simulink model "Maxom_fcs_noncascaded"  (R2025b)
settings: Solver=ode45  StartTime=0.0  StopTime=0.30  FixedStep=1e-6  MaxStep=1e-5  RelTol=1e-4  EnableMultiTasking=on
values from neighbouring files (symbols this model uses):
  Bfric = 0    [PMSMpara.m]
  ffai = 0.008667    [PMSMpara.m]
  Imax = 20    [PMSMpara.m]
  J = 0.044e-4    (= 4.4e-06)    [PMSMpara.m]
  kis = 0    [PMSMpara.m]
  kps = fsc*6.28*J/Kt    (= 0.364364007978)    [PMSMpara.m]
  Kt = np*1.5*ffai    (= 0.0910035)    [PMSMpara.m]
  Ld = Ls    (= 0.00045)    [PMSMpara.m]
  Lq = Ls    (= 0.00045)    [PMSMpara.m]
  np = 7    [PMSMpara.m]
  Rs = 0.5    [PMSMpara.m]
  Tcur = 1/32000    (= 3.125e-05)    [PMSMpara.m]
  Tpwm = 1/32000    (= 3.125e-05)    [PMSMpara.m]
  Tspd = 1/32000    (= 3.125e-05)    [PMSMpara.m]
  wn = 311040    [PMSMpara.m]
  zeta = 1    [PMSMpara.m]
undefined symbols (not defined in the file or in its folder): dspblkCoreblockFVToolHelper, gcbh
libraries: simulink x4, slpidlib x2, spsUniversalBridgeLib x1, spsCurrentMeasurementLib x1, EasyGo_Machine_lib x1, spsPermanentMagnetSynchronousMachineLib x1, spsSVPWMGenerator2LevelLib x1, spsDCVoltageSourceLib x1, sps_lib x1
(part 1 of 4)
Description:
  | %20230207 r13c
  | 版本同 servo_32k_TSMI_r12b_0413ff02mv8_4t9c2cnst
  | 负载转矩前馈滤波截止频率提到1500hz
  | 
  | r13d  模型版本等同 servo_32k_TSMI_r12b_0413ff02mv8_4t11b2
  | 修改速度给定滤波处理逻辑
  | 小改转矩前馈控制系数
settings Model: ModifiedComment=danie -- Wed Jan 05 16:58:37 2022 -- Version 1.4214  ParamWorkspaceSource=ReferencedWorkspace  TunableVars=Comp_curr_lmt,CurrRampTime_s,DT_Comp_curr_lmt,DT_Comp_curr_uplmt,DT_Comp_freq_lmt,DT_Comp_freq_lmt1,DT_Comp_freq_off_lmt,DT_Comp_reg_uplmt,DT_Comp_table_length,DeadTime_comp_mode,DecOVPEn,K_angle_comp,K_obs,Ki_udcctrl_ID,Kp_udcctrl_ID,Kudcctrl,OpenLoopCtrlEn,OvIdLmtMax,OvIdLmtMin,OverVoltLmHi,SPD_RES_EN,Servo_start_mode,SynFailCfmTime_ms,SynFailDetectEnable,Udc,We_Adapt_Max_set,damping_enable,dc_pos_time,dt_comp_curr_table,dt_comp_reg_table,flystr_sc_time,fs_flystart_Hz_set,fw_us_max,idc_pos_ref,idc_pos_time,iq_opnlp_curr_ref,is_opn_max,k_TorqFwd_c1,k_TorqFwd_c2,k_aw,k_emf_cnst_krpm,k_load_torq_comp,k_res_damp1,k_res_damp2,k_we_damp,k_wr_adj,ki_cur_ctrl,ki_flux_wkn,ki_is_load_comp,ki_is_magn_comp,ki_psir_adapt,ki_rs_adapt,ki_spd_ctrl,ki_spd_ctrl_low,ki_we_adapt,ki_wr_est_pll,kp_cur_ctrl,kp_flux_wkn,kp_is_load_comp,kp_is_magn_comp,kp_psir_adapt,kp_rs_adapt,kp_spd_ctrl,kp_spd_ctrl_low,kp_we_adapt,kp_wr_est_pll,ld_calc,lq_calc,maxfreqref_Hz,motor_start_mode,mtr_rated_cur_set,mtr_rated_freq_set,normal_acc_time_s,openloopTest,opnlp_acc_time,pn_calc,psir_calc,rs_calc,sc_test_Imax,spd_ctrl_out_max,spd_ctrl_out_min,startfrqholdtime_s,sw_wr_hi,sw_wr_lo,sw_wr_mag_hi,sw_wr_mag_lo,swtich_freq_spd_ctrl_hi,swtich_freq_spd_ctrl_low,ts_calc_cur_set,ts_calc_obs_set,ts_flystart_set,udc_r,ukf_spd_calc_en,w_startfrq,ws_merge_mode,ws_no_merge  TunableVarsStorageClass=Auto,Auto,Auto,Auto,Auto,Auto,Auto,Auto,Auto,Auto,Auto,Auto,Auto,Auto,Auto,Auto,Auto,Auto,Auto,Auto,Auto,Auto,Auto,Auto,Auto,Auto,Auto,Auto,Auto,Auto,Auto,Auto,Auto,Auto,Auto,Auto,Auto,Auto,Auto,Auto,Auto,Auto,Auto,Auto,Auto,Auto,Auto,Auto,Auto,Auto,Auto,Auto,Auto,Auto,Auto,Auto,Auto,Auto,Auto,Auto,Auto,Auto,Auto,Auto,Auto,Auto,Auto,Auto,Auto,Auto,Auto,Auto,Auto,Auto,Auto,Auto,Auto,Auto,Auto,Auto,Auto,Auto,Auto,Auto,Auto,Auto,Auto,Auto,Auto,Auto,Auto,Auto,Auto,Auto,Auto,Auto  TunableVarsTypeQualifier=,,,,,,,,,,,,,,,,,,,,,,,,,,,,,,,,,,,,,,,,,,,,,,,,,,,,,,,,,,,,,,,,,,,,,,,,,,,,,,,,,,,,,,,,,,,,,,,  VariantFading=off  Creator=MATLAB05  LastModifiedBy=dayanakhegay
settings Model: ModifiedHistory=|
  | danie -- Wed Jan 05 16:58:37 2022 -- Version 1.4214
  | 
  | 
  | danie -- Wed Jan 05 16:58:37 2022 -- Version 1.4214
  | 
  | 
  | danie -- Wed Jan 05 16:44:40 2022 -- Version 1.4213
  | 
  | 
  | danie -- Wed Jan 05 16:23:23 2022 -- Version 1.4212
  | 
  | 
  | danie -- Wed Jan 05 15:12:40 2022 -- Version 1.4211
  | 
  | 
  | danie -- Wed Jan 05 11:32:37 2022 -- Version 1.4208
  | 
  | 
  | danie -- Wed Jan 05 11:32:37 2022 -- Version 1.4208
  | 
  | 
  | danie -- Wed Jan 05 11:32:37 2022 -- Version 1.4208
  | 
  | 
  | danie -- Wed Jan 05 11:32:37 2022 -- Version 1.4208
  | 
  | 
  | danie -- Wed Jan 05 11:32:37 2022 -- Version 1.4208
  | 
  | 
  | danie -- Wed Jan 05 11:32:37 2022 -- Version 1.4208
  | 
  | 
  | danie -- Wed Jan 05 11:32:37 2022 -- Version 1.4208
  | 
  | 
  | danie -- Wed Jan 05 11:32:37 2022 -- Version 1.4208
  | 
  | 
  | danie -- Tue Jan 04 20:01:11 2022 -- Version 1.4189
  | 
  | 
  | danie -- Tue Jan 04 20:01:11 2022 -- Version 1.4189
  | 
  | 
  | danie -- Tue Jan 04 20:01:11 2022 -- Version 1.4189
  | 
  | 
  | danie -- Tue Jan 04 20:01:11 2022 -- Version 1.4189
  | 
  | 
  | danie -- Tue Jan 04 20:01:11 2022 -- Version 1.4189
  | 
  | 
  | danie -- Tue Jan 04 20:01:11 2022 -- Version 1.4189
  | 
  | 
  | danie -- Tue Jan 04 20:01:11 2022 -- Version 1.4189
  | 
  | 
  | danie -- Tue Jan 04 20:01:11 2022 -- Version 1.4189
  | 
  | 
  | danie -- Tue Jan 04 20:01:11 2022 -- Version 1.4189
  | 
  | 
  | danie -- Tue Jan 04 20:01:11 2022 -- Version 1.4189
  | 
  | 
  | danie -- Tue Jan 04 20:01:11 2022 -- Version 1.4189
  | 
  | 
  | danie -- Tue Jan 04 20:01:11 2022 -- Version 1.4189
  | 
  | 
  | danie -- Tue Jan 04 20:01:11 2022 -- Version 1.4189
  | 
  | 
  | danie -- Tue Jan 04 20:01:11 2022 -- Version 1.4189
  | 
  | 
  | danie -- Tue Jan 04 20:01:11 2022 -- Version 1.4189
  | 
  | 
  | danie -- Tue Jan 04 20:01:11 2022 -- Version 1.4189
  | 
  | 
  | danie -- Tue Jan 04 20:01:11 2022 -- Version 1.4189
  | 
  | 
  | danie -- Tue Jan 04 20:01:11 2022 -- Version 1.4189
  | 
  | 
  | danie -- Tue Jan 04 20:01:11 2022 -- Version 1.4189
  | 
  | 
  | danie -- Tue Jan 04 20:01:11 2022 -- Version 1.4189
  | 
  | 
  | danie -- Tue Jan 04 20:01:11 2022 -- Version 1.4189
  | 
  | 
  | danie -- Tue Jan 04 20:01:11 2022 -- Version 1.4189
  | 
  | 
  | danie -- Tue Jan 04 20:01:11 2022 -- Version 1.4189
  | 
  | 
  | danie -- Tue Jan 04 20:01:11 2022 -- Version 1.4189
  | 
  | 
  | danie -- Tue Jan 04 20:01:11 2022 -- Version 1.4189
  | 
  | 
  | danie -- Tue Jan 04 20:01:11 2022 -- Version 1.4189
  | 
  | 
  | danie -- Tue Jan 04 20:01:11 2022 -- Version 1.4189
  | 
  | 
  | danie -- Tue Jan 04 20:01:11 2022 -- Version 1.4189
  | 
  | 
  | danie -- Tue Jan 04 20:01:11 2022 -- Version 1.4189
  | 
  | 
  | danie -- Tue Jan 04 20:01:11 2022 -- Version 1.4189
  | 
  | 
  | danie -- Tue Jan 04 20:01:11 2022 -- Version 1.4189
  | 
  | 
  | danie -- Tue Jan 04 18:06:07 2022 -- Version 1.4188
  | 
  | 
  | danie -- Tue Jan 04 17:34:36 2022 -- Version 1.4187
  | 
  | 
  | danie -- Tue Jan 04 17:26:52 2022 -- Version 1.4186
  | 
  | 
  | danie -- Tue Jan 04 17:22:15 2022 -- Version 1.4185
  | add merge mode 2( time merge mode)
  | 
  | danie -- Tue Jan 04 16:56:47 2022 -- Version 1.4179
  | 
  | 
  | danie -- Tue Jan 04 16:56:47 2022 -- Version 1.4179
  | 
  | 
  | danie -- Tue Jan 04 16:56:47 2022 -- Version 1.4179
  | 
  | 
  | danie -- Tue Jan 04 16:56:47 2022 -- Version 1.4179
  | 
  | 
  | danie -- Tue Jan 04 16:56:47 2022 -- Version 1.4179
  | 
  | 
  | danie -- Tue Jan 04 16:56:47 2022 -- Version 1.4179
  | 
  | 
  | danie -- Tue Jan 04 16:56:47 2022 -- Version 1.4179
  | 
  | 
  | danie -- Tue Jan 04 16:56:47 2022 -- Version 1.4179
  | 
  | 
  | danie -- Tue Jan 04 16:24:52 2022 -- Version 1.4174
  | 
  | 
  | danie -- Tue Jan 04 16:24:52 2022 -- Version 1.4174
  | 
  | 
  | danie -- Tue Jan 04 16:24:52 2022 -- Version 1.4174
  | 
  | 
  | danie -- Tue Jan 04 16:24:52 2022 -- Version 1.4174
  | 
  | 
  | danie -- Tue Jan 04 16:24:52 2022 -- Version 1.4174
  | 
  | 
  | danie -- Tue Jan 04 16:24:52 2022 -- Version 1.4174
  | 
  | 
  | danie -- Tue Jan 04 16:13:51 2022 -- Version 1.4173
  | 
  | try to modify merge（low/high spd）spd fdb logic
  | 
  | danie -- Tue Jan 04 15:54:14 2022 -- Version 1.4172
  | 
  | 
  | danie -- Thu Dec 30 11:22:47 2021 -- Version 1.4171
  | 
  | 
  | danie -- Thu Dec 30 11:13:03 2021 -- Version 1.4170
  | 
  | 
  | danie -- Thu Dec 30 10:44:02 2021 -- Version 1.4167
  | 
  | 
  | danie -- Thu Dec 30 10:44:02 2021 -- Version 1.4167
  | 
  | 
  | danie -- Thu Dec 30 10:44:02 2021 -- Version 1.4167
  | 
  | 
  | danie -- Thu Dec 30 10:37:28 2021 -- Version 1.4166
  | 
  | 
  | danie -- Wed Dec 29 18:47:50 2021 -- Version 1.4165
  | 
  | 
  | danie -- Wed Dec 29 18:47:08 2021 -- Version 1.4164
  | 
  | 优化转矩前馈，和电流指令前馈
  | 修改速度PID模块，
  | 速度环输出加入超前滞后补偿环节
  | 
  | danie -- Tue Dec 28 11:57:05 2021 -- Version 1.4144
  | 
  | 1. fix alig function logic， function code write-back logic debug
  | 2. dec run logic after 2-levle current control（10hz），
  | 3. save eeprom ok
settings SolverCC: AlgebraicLoopSolver=TrustRegion
settings DataIOCC: LimitDataPoints=on  SaveFormat=StructureWithTime  SignalLoggingSaveFormat=ModelDataLogs  DSMLogging=off  ReturnWorkspaceOutputs=off
settings OptimizationCC: DefaultParameterBehavior=Inlined  UseFloatMulNetSlope=on  DefaultUnderspecifiedDataType=single  UseSpecifiedMinMax=on  InlineInvariantSignals=on  ExpressionDepthLimit=2147483647.0  StateBitsets=on  DataBitsets=on  ZeroExternalMemoryAtStartup=off  InitFltsAndDblsToZero=on  EfficientFloat2IntCast=on  EfficientMapNaN2IntZero=off  LifeSpan=1  SimCompilerOptimization=on  EfficientTunableParamExpr=on
settings DebuggingCC: SignalInfNanChecking=warning  SignalRangeChecking=warning  SaveWithParameterizedLinksMsg=none  UnderspecifiedInitializationDetection=Classic  MergeDetectMultiDrivingBlocksExec=none  SignalResolutionControl=TryResolveAllWithWarning  MaxConsecutiveZCsMsg=none  SolverPrmCheckMsg=warning  CheckMatrixSingularityMsg=warning  ParameterPrecisionLossMsg=none  ParameterTunabilityLossMsg=none  UnconnectedInputMsg=warning  UnconnectedOutputMsg=warning  UnconnectedLineMsg=warning  AllowSymbolicDim=off  StateNameClashWarn=warning  SFUnexpectedBacktrackingDiag=warning  SFNoUnconditionalDefaultTransitionDiag=warning  SFExecutionAtInitializationDiag=none  ArithmeticOperatorsInVariantConditions=warning
settings HardwareCC: ProdBitPerPointer=32.0  ProdBitPerSizeT=32.0  ProdBitPerPtrDiffT=32.0  ProdLargestAtomicInteger=Long  ProdLargestAtomicFloat=Double  ProdWordSize=32.0  ProdLongLongMode=on  ProdHWDeviceType=ARM Compatible->ARM Cortex  TargetBitPerLong=64.0  TargetBitPerPointer=64.0  TargetBitPerSizeT=64.0  TargetBitPerPtrDiffT=64.0  TargetLongLongMode=on  TargetIntDivRoundTo=Zero  TargetEndianess=LittleEndian  TargetWordSize=64.0  TargetHWDeviceType=MATLAB Host  ProdEqTarget=off
settings ModelReferenceCC: EnableRefExpFcnMdlSchedulingChecks=on  PropagateSignalLabelsOutOfModel=off
settings SFSimCC: SimUseLocalCustomCode=off  MATLABDynamicMemAlloc=off  CustomCodeUndefinedFunction=UseInterfaceOnly
settings RTWCC: SystemTargetFile=ert.tlc  GenCodeOnly=on  TemplateMakefile=ert_default_tmf  GenerateReport=on  RTWUseLocalCustomCode=off  BuildConfiguration=Faster Runs  IncludeHyperlinkInReport=on  LaunchReport=on  GenerateTraceInfo=on  GenerateTraceReport=on  GenerateTraceReportSl=on  GenerateTraceReportSf=on  GenerateTraceReportEml=on  GPUComputeCapability=3.5  Description=Embedded Coder
settings RTWCC: CustomInclude=|
  | ..\..\
  | ..\..\FuncodeFile
  | ..\..\MotorCtrl\inc
  | ..\..\Common\inc
  | ..\..\IQmath_to_CMSIS\include
settings CodeAppCC: IgnoreCustomStorageClasses=off  StateflowObjectComments=on  MATLABSourceComments=on
settings ERTTargetCC: InlinedParameterPlacement=Hierarchical  ERTCustomFileTemplate=example_file_process.tlc  SuppressUnreachableDefaultCases=off  MemSecPackage=mpt  DynamicArrayContainerType=coder::array  TargetLangStandard=C99 (ISO)  MultiwordLength=2048.0  GenerateSampleERTMain=on  IncludeMdlTerminateFcn=off  CombineSignalStateStructs=on  SuppressErrorStatus=on  SupportAbsoluteTime=off  SupportNonFinite=off
settings ConfigComp: CovMetricSettings=dw  CovSaveCumulativeToWorkspaceVar=on  CovSaveSingleToWorkspaceVar=on  CovExternalEMLEnable=off  CovSFcnEnable=off  PSEnableModelRefIgnoreList=off  PSModelRefMinMaxVerif=CheckAndConstrain  PSAutoStubLUT=off
settings SimscapeCC: SimscapeNormalizeSystem=off

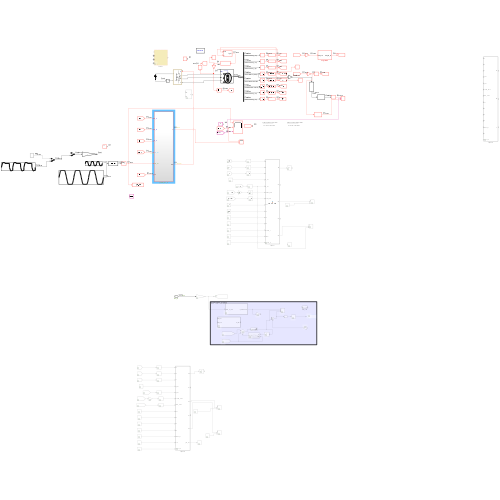
[thumbnail: Simulink's stored preview of the top-level diagram]
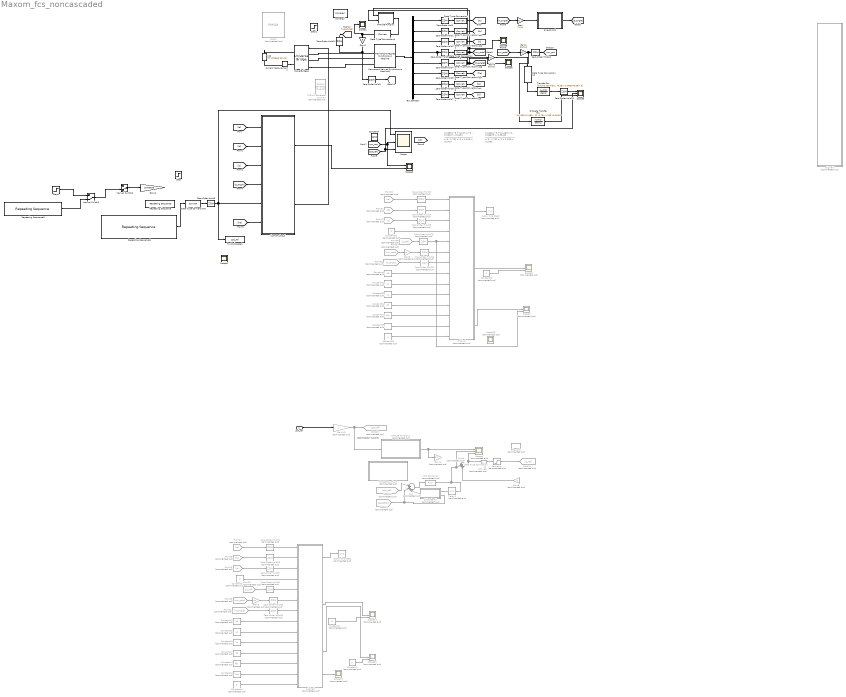
== system Maxom_fcs_noncascaded ==
  note: 0.1206 z^3 + 0.1469 z^2 - 0.06819 z - 0.09442
      | ---------------------------------------------
      | z^3 - 1.761 z^2 + 1.109 z - 0.2432
  note: 0.1038 z^3 + 0.2274 z^2 - 0.1843 z - 0.0451
      | -------------------------------------------
      | z^3 - 1.761 z^2 + 1.105 z - 0.2414
  note: 速度环控制器+电流前馈
  spd_ref : Inport
  2levelBridge1 : spsUniversalBridgeLib/Universal Bridge  Arms=3  SnubberResistance=1e5  SnubberCapacitance=inf  Device=MOSFET / Diodes  Ron=1e-3  Lon=0  ForwardVoltages="[  0  0  ]"  ForwardVoltage=0  GTOparameters=[ 10e-6 , 20e-6 ]  IGBTparameters=[ 1e-6 , 2e-6 ]  Measurements=None  Measurements_2=None  converterType=Rectifier
  Bus Selector : BusSelector  OutputSignals=Stator current is_a (A),Stator current is_b (A),Stator current is_c (A),Rotor speed wm (rad/s),Rotor angle thetam (rad),Electromagnetic torque Te (N*m),Stator current is_q (A),Stator current is_d (A)
  Constant{10..11,31,47} (4 alike) : Constant  Commented=on  Value=0
  Constant2 : Constant  Commented=on  Value=5
  Constant32 : Constant  Commented=on  Value=Ld
  Constant33 : Constant  Commented=on  Value=Lq
  Constant34 : Constant  Commented=on  Value=Rs
  Constant35 : Constant  Commented=on  Value=Tpwm
  Constant36 : Constant  Commented=on  Value=2
  Constant37 : Constant  Commented=on  Value=ffai
  Constant39 : Constant  Commented=on  Value=Ld
  Constant40 : Constant  Commented=on  Value=Lq
  Constant41 : Constant  Commented=on  Value=Rs
  Constant42 : Constant  Commented=on  Value=Tcur
  Constant43 : Constant  Commented=on  Value=3
  Constant44 : Constant  Commented=on  Value=ffai
  Constant45 : Constant  Commented=on  Value=48
  Constant7 : Constant  Value=2000  OutDataTypeStr=single
  Constant8 : Constant  Commented=on  Value=48
  Current Measurement1 : spsCurrentMeasurementLib/Current Measurement  PhasorSimulation=off  OutputType=Complex  PSBequivalent=0
  Data Type Conversion{,1..10} (11 alike) : DataTypeConversion  SaturateOnIntegerOverflow=off  RndMeth=Floor
  Data Type Conversion11 : DataTypeConversion  Commented=on  SaturateOnIntegerOverflow=off  RndMeth=Floor
  Delay One Step1 : Delay  Commented=on  DelayLength=1  SampleTime=1/32000
  Delay One Step3 : Delay  Commented=on  DelayLength=1  SampleTime=1/16000
  Delay1 : Delay  Commented=on  DelayLength=1  InitialCondition=0  SampleTime=Tspd
  Discrete Transfer Fcn : DiscreteTransferFcn  LoadFcn=dspblkCoreblockFVToolHelper(gcbh,'load');  Numerator=[0.1206 0.1469 -0.06819 -0.09442]  Denominator=[1 -1.761 1.109 -0.2432]
      settings: CopyFcn=dspblkCoreblockFVToolHelper(gcbh,'copy');  DeleteFcn=dspblkCoreblockFVToolHelper(gcbh,'close');  ModelCloseFcn=dspblkCoreblockFVToolHelper(gcbh,'close');  PreSaveFcn=dspblkCoreblockFVToolHelper(gcbh,'presave');  PostSaveFcn=dspblkCoreblockFVToolHelper(gcbh,'postsave');  CloseFcn=dspblkCoreblockFVToolHelper(gcbh,'close');
  Filter_13k : Subsystem  Tag=FilterWizardSubSystem  Commented=on
      settings: ErrorFcn=dspFilterRealizedInBasicElemsAlgLoopErrFcnCallback
  From10 : From  Commented=on  GotoTag=spd_ESO
  From13 : From  Commented=on  GotoTag=spd_ref
  From16 : From  Commented=on  GotoTag=ic
  From26 : From  Commented=on  GotoTag=ic
  From27 : From  Commented=on  GotoTag=ia
  From28 : From  Commented=on  GotoTag=ib
  From29 : From  Commented=on  GotoTag=wm_rads
  From30 : From  Commented=on  GotoTag=ia
  From31 : From  Commented=on  GotoTag=ib
  From32 : From  Commented=on  GotoTag=m_angle
  From33 : From  Commented=on  GotoTag=iq_ref
  From34 : From  Commented=on  GotoTag=wm_rads
  From35 : From  Commented=on  GotoTag=m_angle
  From36 : From  Commented=on  GotoTag=iq_ref
  Gain : Gain  Gain=7/2/pi
  Gain1 : Gain  Gain=60/2/pi
  Gain2 : Gain  Gain=3
  Gain26 : Gain  Commented=on
  Gain3 : Gain  Gain=60/2/pi
  Gain4 : Gain  Commented=on  Gain=0.2
  Gain5 : Gain  Commented=on  Gain=np
  Gain6 : Gain  Gain=19.89436
  Gain8 : Gain  Commented=on  Gain=-1
  Gain9 : Gain  Commented=on  Gain=np
  Goto13 : Goto  Commented=on  GotoTag=spd_ref
  Goto14 : Goto  Commented=on  GotoTag=iq_ref
  MATLAB Function : MATLAB Function  TreatAsAtomicUnit=on
  MATLAB Function1 : MATLAB Function  Commented=on  TreatAsAtomicUnit=on
  MATLAB Function3 : MATLAB Function  Commented=on  TreatAsAtomicUnit=on
  Manual Switch2 : ManualSwitch  CurrentSetting=0
  Manual Switch6 : ManualSwitch  CurrentSetting=0
  PID Controller : slpidlib/PID Controller  Commented=on  Controller=PI  Form=Parallel  TimeDomain=Discrete-time  UseExternalTs=off  SampleTime=1/32000  IntegratorMethod=Forward Euler  FilterMethod=Forward Euler  ControllerParametersSource=internal  P=0.044e-4*2*pi*2500*2.05  I=0.0001*4.5*0.2*10  UseKiTs=off  D=0  UseExternalDerivativeSource=off  N=100  UseFilter=on  TunerSelectOption=Transfer Function Based (PID Tuner App)  InitialConditionSource=internal  InitialConditionForIntegrator=0  InitialConditionForFilter=0  DifferentiatorICPrevScaledInput=0  ExternalReset=none  TrackingMode=off  Kt=1  LimitOutput=on  SatLimitsSource=internal  UpperSaturationLimit=20  LowerSaturationLimit=-20  LinearizeAsGain=on  AntiWindupMode=clamping  Kb=0.1  LimitIntegrator=off  UpperIntegratorSaturationLimit=20  LowerIntegratorSaturationLimit=-20  POutMin=[]  POutMax=[]  IOutMin=[]  IOutMax=[]  DOutMin=[]  DOutMax=[]  NOutMin=[]  NOutMax=[]  SumOutMin=[]  SumOutMax=[]  SaturationOutMin=[]  SaturationOutMax=[]  PParamMin=[]  PParamMax=[]  IParamMin=[]  IParamMax=[]  DParamMin=[]  DParamMax=[]  NParamMin=[]  NParamMax=[]  KbParamMin=[]  KbParamMax=[]  KtParamMin=[]  KtParamMax=[]  KbOutMin=[]  KbOutMax=[]  KtOutMin=[]  KtOutMax=[]  IntegratorOutMin=[]  IntegratorOutMax=[]  FilterOutMin=[]  FilterOutMax=[]  SumI1OutMin=[]  SumI1OutMax=[]  SumI2OutMin=[]  SumI2OutMax=[]  SumI3OutMin=[]  SumI3OutMax=[]  SumI4OutMin=[]  SumI4OutMax=[]  SumDOutMin=[]  SumDOutMax=[]  DifferentiatorOutMin=[]  DifferentiatorOutMax=[]  FilterDiffOutCoefMin=[]  FilterDiffOutCoefMax=[]  ReciprocalOutMin=[]  ReciprocalOutMax=[]  SumDenOutMin=[]  SumDenOutMax=[]  SumNumOutMin=[]  SumNumOutMax=[]  DivideOutMin=[]  DivideOutMax=[]  UdiffTsProdOutMin=[]  UdiffTsProdOutMax=[]  NTsProdOutMin=[]  NTsProdOutMax=[]  UintegralTsProdOutMin=[]  UintegralTsProdOutMax=[]  UngainTsProdOutMin=[]  UngainTsProdOutMax=[]  ClampingZeroOutDataTypeStr=Inherit: Inherit via back propagation  ClampingZeroOutMin=[]  ClampingZeroOutMax=[]  FilterDenConstantOutDataTypeStr=Inherit: Inherit via back propagation  FilterDenConstantOutMin=[]  FilterDenConstantOutMax=[]  PCopyOutDataTypeStr=Inherit: Inherit via back propagation  PCopyOutMin=[]  PCopyOutMax=[]  NCopyOutDataTypeStr=Inherit: Inherit via back propagation  NCopyOutMin=[]  NCopyOutMax=[]  IntegratorContinuousStateAttributes=''  IntegratorStateMustResolveToSignalObject=off  IntegratorRTWStateStorageClass=Auto  FilterContinuousStateAttributes=''  FilterStateMustResolveToSignalObject=off  FilterRTWStateStorageClass=Auto  ParallelPVariant=InternalParameters  IdealPVariant=Disabled  IVariant=InternalParameters  DVariant=Disabled  IntegratorVariant=Discrete  SatVariant=Enabled  AWVariant=DiscClampingParallel  PCopyVariant=Disabled  TRVariant=Disabled  FdbkBlocksVariant=Forward  IdealPFdbkVariant=Disabled  SatFdbkVariant=Disabled  DerivativeFilterVariant=Disabled  NVariant=Disabled  NCopyVariant=Disabled_SignalSpec  FilterICVariant=Disabled  IntegratorICVariant=InternalICs  ExternalResetVariant=Disabled  TRSumVariant=Passthrough  SumFdbkVariant=Disabled  SumVariant=Sum_PI  TsampFilterVariant=InternalTs  TsampNgainVariant=Passthrough  TsampIntegralVariant=Disabled_SignalSpec  ExternalSaturationOutDataTypeStr=Inherit: Same as second input  DerivativeSourceVariant=Disabled  PreIntVariant=InternalPreInt
  PMSM : EasyGo_Machine_lib/Commonly Used Motor/PMSM  Commented=on  LabelModeActiveChoice=TST  MechanicalLoad=Torque Tm  RotorType=Salient-pole  Resistance=0.5  La=0.000395  dqInductances=[0.45e-3, 0.48e-3]  MachineConstant=Torque constant (N.m/A_peak)  Flux=0.1318  VoltageCst=35  TorqueCst=0.091003  Mechanical=[0.044e-4*2 0.000000 7 0]  PolePairs=4  useencoder=on  CN_E=Connector 2  DO_encoder=[8,9,10]  encoderpulses=2500  Zphase=0  usehall=off  CN_H=Connector 1  DO_hall=[3,4,5]  hallphase=0  useresolver=on  CN_R_AO=Connector 1  AO=[0,1]  gain_ao=[1,1]  offset_ao=[0,0]  CN_R_AI=Connector 1  AI=0  gain_ai=1  offset_ai=0  pairs=4  Angle=0
      link override TSV/PMSM: RefAngle=90 degrees behind phase A axis (modified Park)
      settings: SourceProductName=EasyGo Machine
  Permanent Magnet Synchronous Machine2 : spsPermanentMagnetSynchronousMachineLib/Permanent Magnet Synchronous Machine  NbPhases=3  FluxDistribution=Sinusoidal  RotorType=Salient-pole  MechanicalLoad=Torque Tm  PresetModel=No  ShowDetailedParameters=on  MeasurementBus=off  Resistance=Rs  Inductance=8.5e-3  dqInductances=[Ld,Lq]  La=Ld  MachineConstant=Torque Constant (N.m / A_peak)  Flux=0.008667  VoltageCst=11.0041  TorqueCst=Kt  Flat=150  Mechanical=[J*4 0 np 0]  PolePairs=np  InitialConditions=[0, 0, 0,0]  InitialConditions5ph=[0 0 0 0 0 0]  RefAngle=90 degrees behind phase A axis (modified Park)  IterativeDiscreteModel=Trapezoidal non iterative  TsBlock=-1  TsPowergui=0
  Repeating Sequence : simulink/Sources/Repeating Sequence  rep_seq_t=[0 0.001 0.004 0.006 0.009 0.01]  rep_seq_y=[0 990 990 -990 -990 0]
  Repeating Sequence1 : simulink/Sources/Repeating Sequence  rep_seq_t=[0 3.125e-05 6.25e-05 9.375e-05 0.000125 0.00015625 0.0001875 0.00021875 0.00025 0.00028125 0.0003125 0.00034375 0.000375 0.00040625 0.0004375 0.00046875 0.0005 0.00053125 0.0005625 0.00059375 0.000625 0.00065625 0.0006875 0.00071875 0.00075 0.00078125 0.0008125 0.00084375 0.000875 0.00090625 0.0009375 0.00096875 0.001 0.00103125 0.0010625 0.00109375 0.001125 0.00115625 0.0011875 0.00121875 0.00125 0.00128125 0.0013125 0.00134375 0.001375 0.00140625 0.0014375 0.00146875 0.0015 0.00153125 0.0015625 0.00159375 0.001625 0.00165625 0.0016875 0.00171875 0.00175 0.00178125 0.0018125 0.00184375 0.001875 0.00190625 0.0019375 0.00196875 0.002 0.00203125 0.0020625 0.00209375 0.002125 0.00215625 0.0021875 0.00221875 0.00225 0.00228125 0.0023125 0.00234375 0.002375 0.00240625 0.0024375 0.00246875 0.0025 0.00253125 0.0025625 0.00259375 0.002625 0.00265625 0.0026875 0.00271875 0.00275 0.00278125 0.0028125 0.00284375 0.002875 0.00290625 0.0029375 0.00296875 0.003 0.00303125 0.0030625 0.00309375 0.003125 0.00315625 0.0031875 0.00321875 0.00325 0.00328125 0.0033125 0.00334375 0.003375 0.00340625 0.0034375 0.00346875 0.0035 0.00353125 0.0035625 0.00359375 0.003625 0.00365625 0.0036875 0.00371875 0.00375 0.00378125 0.0038125 0.00384375 0.003875 0.00390625 0.0039375 0.00396875 0.004 0.00403125 0.0040625 0.00409375 0.004125 0.00415625 0.0041875 0.00421875 0.00425 0.00428125 0.0043125 0.00434375 0.004375 0.00440625 0.0044375 0.00446875 0.0045 0.00453125 0.0045625 0.00459375 0.004625 0.00465625 0.0046875 0.00471875 0.00475 0.00478125 0.0048125 0.00484375 0.004875 0.00490625 0.0049375 0.00496875 0.005 0.00503125 0.0050625 0.00509375 0.005125 0.00515625 0.0051875 0.00521875 0.00525 0.00528125 0.0053125 0.00534375 0.005375 0.00540625 0.0054375 0.00546875 0.0055 0.00553125 0.0055625 0.00559375 0.005625 0.00565625 0.0056875 0.00571875 0.00575 0.00578125 0.0058125 0.00584375 0.005875 0.00590625 0.0059375 0.00596875 0.006 0.00603125 0.0060625 0.00609375 0.006125 0.00615625 0.0061875 0.00621875 0.00625 0.00628125 0.0063125 0.00634375 0.006375 0.00640625 0.0064375 0.00646875 0.0065 0.00653125 0.0065625 0.00659375 0.006625 0.00665625 0.0066875 0.00671875 0.00675 0.00678125 0.0068125 0.00684375 0.006875 0.00690625 0.0069375 0.00696875 0.007 0.00703125 0.0070625 0.00709375 0.007125 0.00715625 0.0071875 0.00721875 0.00725 0.00728125 0.0073125 0.00734375 0.007375 0.00740625 0.0074375 0.00746875 0.0075 0.00753125 0.0075625 0.00759375 0.007625 0.00765625 0.0076875 0.00771875 0.00775 0.00778125 0.0078125 0.00784375 0.007875 0.00790625 0.0079375 0.00796875 0.008 0.00803125 0.0080625 0.00809375 0.008125 0.00815625 0.0081875 0.00821875 0.00825 0.00828125 0.0083125 0.00834375 0.008375 0.00840625 0.0084375 0.00846875 0.0085 0.00853125 0.0085625 0.00859375 0.008625 0.00865625 0.0086875 0.00871875 0.00875 0.00878125 0.0088125 0.00884375 0.008875 0.00890625 0.0089375 0.00896875 0.009 0.00903125 0.0090625 0.00909375 0.009125 0.00915625 0.0091875 0.00921875 0.00925 0.00928125 0.0093125 0.00934375 0.009375 0.00940625 0.0094375 0.00946875 0.0095 0.00953125 0.0095625 0.00959375 0.009625 0.00965625 0.0096875 0.00971875 0.00975 0.00978125 0.0098125 0.00984375 0.009875 0.00990625 0.0099375 0.00996875]  rep_seq_y=[-1.37291121482849;29.5645885467529;60.5020866394043;91.4395980834961;122.377082824707;153.314575195312;184.252090454102;215.189544677734;246.127090454102;277.064544677734;308.002105712891;338.939514160156;369.877075195312;400.814544677734;431.658996582031;462.379089355469;492.935882568359;523.281066894531;553.35693359375;583.094970703125;612.415710449219;641.229309082031;669.435668945312;696.926818847656;723.588195800781;749.302062988281;773.950378417969;797.419372558594;819.603149414062;840.408325195312;859.757202148438;877.591613769531;893.875854492188;908.597534179688;921.769409179688;933.426696777344;943.627990722656;952.450256347656;959.987426757812;966.345336914062;971.637573242188;975.982238769531;979.497192382812;982.296936035156;984.489501953125;986.1748046875;987.442993164062;988.373352050781;989.034118652344;989.483581542969;989.769653320312;989.931396484375;990.000061035156;990.000061035156;990.000061035156;990.000061035156;990.000061035156;990.000061035156;990.000061035156;990.000061035156;990.000061035156;990.000061035156;990;990;990;990;990;989.999938964844;990;989.999938964844;989.999938964844;989.999938964844;989.999938964844;989.999938964844;989.999938964844;990;990;990;989.999938964844;989.999877929688;990;990.000061035156;990.000061035156;990.000183105469;990.000183105469;990.000183105469;990.000183105469;990.000183105469;990.000183105469;990.000122070312;990.000061035156;990.000061035156;990;990;990;990;990;990;990;990;990;990;989.999938964844;989.999938964844;989.999938964844;990;990;990;990;990;989.906921386719;989.689575195312;989.308837890625;988.716735839844;987.85498046875;986.655639648438;985.038818359375;982.914794921875;980.183715820312;976.737426757812;972.461364746094;967.237670898438;960.948364257812;953.479736328125;944.726196289062;934.593688964844;923.004943847656;909.901794433594;895.248840332031;879.033142089844;861.267395019531;841.987060546875;821.250732421875;799.135559082031;775.735168457031;751.155395507812;725.510192871094;698.917602539062;671.495056152344;643.357299804688;614.612243652344;585.360290527344;555.69091796875;525.68359375;495.407073974609;464.918975830078;434.267517089844;403.491790771484;372.622863769531;341.685424804688;310.747924804688;279.810394287109;248.872909545898;217.935424804688;186.997909545898;156.060394287109;125.122909545898;94.185417175293;63.2479095458984;32.3104095458984;1.37291896343231;-29.5645847320557;-60.5020942687988;-91.439582824707;-122.377052307129;-153.314544677734;-184.252090454102;-215.189544677734;-246.127090454102;-277.064575195312;-308.002136230469;-338.939514160156;-369.877075195312;-400.814544677734;-431.659027099609;-462.379089355469;-492.935821533203;-523.281005859375;-553.356994628906;-583.094909667969;-612.415710449219;-641.229370117188;-669.435791015625;-696.926879882812;-723.588256835938;-749.302185058594;-773.950500488281;-797.41943359375;-819.603271484375;-840.408325195312;-859.757141113281;-877.591552734375;-893.875732421875;-908.597595214844;-921.769348144531;-933.426696777344;-943.627868652344;-952.4501953125;-959.987365722656;-966.345092773438;-971.637390136719;-975.982116699219;-979.497192382812;-982.296875;-984.489440917969;-986.174743652344;-987.442993164062;-988.373352050781;-989.0341796875;-989.483703613281;-989.769775390625;-989.931579589844;-990.000244140625;-990.000244140625;-990.000244140625;-990.000244140625;-990.000244140625;-990.000183105469;-990.000122070312;-990.000122070312;-990.000061035156;-990.000061035156;-990.000061035156;-990.000061035156;-990.000061035156;-990.000061035156;-990.000061035156;-990.000061035156;-990.000061035156;-990.000061035156;-990.000061035156;-990.000061035156;-990.000061035156;-990.000061035156;-990.000061035156;-990.000061035156;-990.000061035156;-990;-990;-990;-990;-990;-990;-990;-990;-990;-989.999938964844;-989.999938964844;-989.999938964844;-990;-990;-990;-990;-990;-990.000061035156;-990.000122070312;-990.000122070312;-990.000183105469;-990.000183105469;-990.000244140625 ...(+1076 chars)]
  Repeating Sequence3 : simulink/Sources/Repeating Sequence  rep_seq_t=[0 1e-3 3e-3 3.1e-3 7e-3 7.1e-3 8.1e-3 9e-3 9.1e-3 10e-3]  rep_seq_y=[0 65 65 55 55 0 -45 -45 -40 -40]
  SVPWM Generator (2-Level) : spsSVPWMGenerator2LevelLib/SVPWM Generator (2-Level)  Commented=on  InputType=alpha-beta components  SwitchingPattern=Pattern #1  Fc=16000  ParUref=[0.8 -30 50]  Ts=0
  Saturation : Saturate  Commented=on  UpperLimit=20  LowerLimit=-20
  Scope : Scope  NumInputPorts=3
      settings: ActiveDisplayYMinimum=-1116.4749751817312  ActiveDisplayYMaximum=1639.1640629042063
  Scope{1..2,6,9} (4 alike) : Scope
      Scope1 settings: ActiveDisplayYMinimum=-1  ActiveDisplayYMaximum=1  DataLoggingVariableName=ScopeData4
      Scope2 settings: ActiveDisplayYMinimum=-1318.9439071765489  ActiveDisplayYMaximum=1431.3010261069821  DataLoggingVariableName=ScopeData3
      Scope6 settings: ActiveDisplayYMinimum=-1  ActiveDisplayYMaximum=1  DataLoggingVariableName=ScopeData16
      Scope9 settings: ActiveDisplayYMinimum=-1  ActiveDisplayYMaximum=1  DataLoggingVariableName=ScopeData19
  Scope13 : Scope  Commented=on
      settings: ActiveDisplayYMinimum=-3.9999999999999991  ActiveDisplayYMaximum=36  DataLoggingVariableName=ScopeData23
  Scope{4..5,7,14..15} (5 alike) : Scope  Commented=on  NumInputPorts=3
      Scope14 settings: ActiveDisplayYMinimum=-12.5593891879434  ActiveDisplayYMaximum=2.9425039784674558  DataLoggingVariableName=ScopeData24
      Scope15 settings: ActiveDisplayYMinimum=-105.05278530395582  ActiveDisplayYMaximum=102.98544731831397  DataLoggingVariableName=ScopeData25
      Scope4 settings: ActiveDisplayYMinimum=-0.36726872757215823  ActiveDisplayYMaximum=1.8083687968233839  DataLoggingVariableName=ScopeData14
      Scope5 settings: ActiveDisplayYMinimum=-43.463268606334395  ActiveDisplayYMaximum=98.317221994212  DataLoggingVariableName=ScopeData15
      Scope7 settings: ActiveDisplayYMinimum=-81.673548802110432  ActiveDisplayYMaximum=106.83519262970458  DataLoggingVariableName=ScopeData17
  Scope19 : Scope  Commented=on
      settings: ActiveDisplayYMinimum=-69.9108444755679  ActiveDisplayYMaximum=52.561016878458716  DataLoggingVariableName=ScopeData29
  Scope3 : Scope  NumInputPorts=3
      settings: ActiveDisplayYMinimum=1508.6642090637922  ActiveDisplayYMaximum=2308.9101103411604  DataLoggingVariableName=ScopeData5
  Scope8 : Scope  NumInputPorts=2
      settings: ActiveDisplayYMinimum=-2576.7416687011719  ActiveDisplayYMaximum=2473.8097839355469  DataLoggingVariableName=ScopeData18
  Step : Step  Time=4096/32000  Before=2000  After=-2000  OutDataTypeStr=single  SampleTime=1/32000
  Step1 : Step  Time=200/32000  After=0.05  SampleTime=1/32000
  Step2 : Step  Time=0.01  After=60  SampleTime=0
  Subsystem3 : Subsystem  Commented=on
  Sum : Sum  Commented=on  Inputs=|+--
  Sum6 : Sum  Commented=on  Inputs=|+++
  To Workspace1 : ToWorkspace  VariableName=spd_ref  SaveFormat=Timeseries  SampleTime=1/32000
  Transfer Fcn : TransferFcn  Numerator=[(1+2*0.707)*(3000*6.28)^2,(3000*6.28)^3]  Denominator=[1 (1+2*0.707)*(3000*6.28) (1+2*0.707)*(3000*6.28)^2 (3000*6.28)^3]
  Vdc : spsDCVoltageSourceLib/DC Voltage Source  Amplitude=48  Measurements=None
  Zero-Order Hold{,1..7,9..12} (12 alike) : ZeroOrderHold  SampleTime=1/32000
  Zero-Order Hold{13..18} (6 alike) : ZeroOrderHold  Commented=on  SampleTime=Tpwm
  Zero-Order Hold{32..37} (6 alike) : ZeroOrderHold  Commented=on  SampleTime=Tcur
  Zero-Order Hold8 : ZeroOrderHold  SampleTime=Tpwm
  ang_comp2 : MATLAB Function  TreatAsAtomicUnit=on
  f_pmsm_foc_sl : Subsystem
  original : MATLAB Function  Commented=on  TreatAsAtomicUnit=on
  original2 : MATLAB Function  Commented=on  TreatAsAtomicUnit=on
  original3 : MATLAB Function  Commented=on  TreatAsAtomicUnit=on
  powergui : sps_lib/powergui  Priority=1  SimulationMode=Continuous  SampleTime=Tcur/20  frequency=60  Iterations=50  frequencyindice=0  Pbase=100e6  ErrMax=1e-4  UnitsV=kV  UnitsW=MW  buscounter=0  FunctionMessages=off  echomessages=off  EnableUseOfTLC=off  CurrentSourceSwitches=off  DisableSnubberDevices=off  DisableRonSwitches=off  DisableVfSwitches=off  DisplayEquations=off  AutomaticDiscreteSolvers=off  SolverType=Tustin/Backward Euler (TBE)  Interpol=off  ExternalGateDelay=off  methode=off  Ts=10  x0status=blocks  SPID=off  SwTol=0  HookPort=off  NonlinearTolerance=1e-4  nMaxIteration=100  ContinueOnMaxIteration=off  RestoreLinks=warning  ResistiveCurrentMeasurement=off  Frange=[0:2:500]  Ylog=off  Xlog=on  ShowGrid=off  save=off  variable=ZData  structure=0  ZoomFFT=off  StartTime=0.0  cycles=1  DisplayStyle=1  fundamental=60  FreqAxis=off  MaxFrequency=1000  frequencyindicesteady=1  RmsSteady=1  display=off
  tag scope: T_load_real=global, real_load=global, wm_rpm=global
  wires:
  Bus Selector/1 -> Zero-Order Hold/1  "<Stator current is_a (A)>"
  Bus Selector/2 -> Zero-Order Hold1/1  "<Stator current is_b (A)>"
  Bus Selector/3 -> Zero-Order Hold2/1  "<Stator current is_c (A)>"
  Bus Selector/4 -> Gain3/1, Zero-Order Hold3/1  "<Rotor speed wm (rad/s)>"
  Bus Selector/7 -> Zero-Order Hold6/1  "<Stator current is_q (A)>"
  Bus Selector/8 -> Zero-Order Hold7/1  "<Stator current is_d (A)>"
  Bus Selector/5 -> Zero-Order Hold4/1  "<Rotor angle thetam (rad)>"
  Bus Selector/6 -> Zero-Order Hold5/1  "<Electromagnetic torque Te (N*m)>"
  Zero-Order Hold/1 -> Data Type Conversion/1
  Zero-Order Hold1/1 -> Data Type Conversion1/1
  Zero-Order Hold2/1 -> Data Type Conversion2/1
  Zero-Order Hold3/1 -> Data Type Conversion3/1
  Zero-Order Hold4/1 -> Data Type Conversion4/1
  Zero-Order Hold5/1 -> Data Type Conversion5/1
  Zero-Order Hold6/1 -> Data Type Conversion6/1
  Zero-Order Hold7/1 -> Data Type Conversion7/1
  [ia] -> f_pmsm_foc_sl/1(Is_A)
  [ib] -> f_pmsm_foc_sl/2(Is_B)
  [ic] -> f_pmsm_foc_sl/3(Is_C)
  [m_angle] -> Gain/1
  Gain/1 -> ang_comp2/1(real_ang)
  ang_comp2/1(real_ang_pu) -> [e_angle]
  [e_angle] -> f_pmsm_foc_sl/4(ang_enc)
  [spd_ref] -> Scope3/2, Scope/3
  [wm_rads] -> Gain1/1
  Gain1/1 -> Discrete Transfer Fcn/1, Zero-Order Hold10/1
  Data Type Conversion/1 -> [ia]
  Data Type Conversion1/1 -> [ib]
  Data Type Conversion2/1 -> [ic]
  Data Type Conversion3/1 -> Scope9/1, MATLAB Function/2(w), [wm_rads]
  Data Type Conversion4/1 -> MATLAB Function/1(theta), Scope6/1, [m_angle]
  Data Type Conversion5/1 -> [Te]
  Data Type Conversion6/1 -> [iq]
  Data Type Conversion7/1 -> [id]
  Data Type Conversion8/1 -> Zero-Order Hold8/1
  Zero-Order Hold8/1 -> To Workspace1/1, f_pmsm_foc_sl/5(spd_ref), Scope/1
  MATLAB Function/1(T_dist) -> Data Type Conversion9/1
  Data Type Conversion9/1 -> Scope1/1, Gain2/1
  Gain2/1 -> Zero-Order Hold11/1, Zero-Order Hold9/1
  Zero-Order Hold9/1 -> [real_load]
  Zero-Order Hold10/1 -> [wm_rpm]
  [wm_rpm] -> Scope8/1, Scope/2
  Transfer Fcn/1 -> Zero-Order Hold12/1
  Data Type Conversion10/1 -> Transfer Fcn/1
  Zero-Order Hold12/1 -> Scope3/1
  Gain3/1 -> Data Type Conversion10/1
  Discrete Transfer Fcn/1 -> Scope3/3
  Zero-Order Hold11/1 -> [T_load_real]
  Permanent Magnet Synchronous Machine2/1 -> Bus Selector/1
  From34/1 -> Gain5/1
  From31/1 -> Zero-Order Hold14/1
  From30/1 -> Zero-Order Hold13/1
  Zero-Order Hold14/1 -> original/2(ib)
  Constant32/1 -> original/9(Ld)
  Constant37/1 -> original/12(lambda_f)
  Zero-Order Hold15/1 -> Scope7/3, original/5(iq_ref)
  Constant33/1 -> original/10(Lq)
  Zero-Order Hold13/1 -> original/1(ia)
  Constant34/1 -> original/11(Rs)
  Constant8/1 -> original/8(Vdc)
  Constant31/1 -> original/4(id_ref)
  Constant35/1 -> original/13(Tpwm)
  spd_ref/1 -> Gain26/1
  Delay1/1 -> Subsystem3/1(iq)
  Gain26/1 -> MATLAB Function1/1(speed_ref_cmd), Goto13/1
  PID Controller/1 -> Scope4/2, Sum6/2, Delay1/1
  Sum6/1 -> Data Type Conversion11/1, Scope4/3
  Gain8/1 -> Sum6/3
  Sum/1 -> PID Controller/1
  MATLAB Function1/1(iq_feedforward) -> Gain4/1, Scope4/1
  From10/1 -> Subsystem3/2(spd), Sum/2
  Subsystem3/1(smt_err) -> Sum/3
  From13/1 -> Sum/1
  Data Type Conversion11/1 -> Saturation/1
  Saturation/1 -> Goto14/1
  Gain5/1 -> Zero-Order Hold16/1
  From35/1 -> Zero-Order Hold17/1
  From16/1 -> Zero-Order Hold18/1
  Constant10/1 -> Scope5/3
  Zero-Order Hold18/1 -> original/3(ic)
  Zero-Order Hold16/1 -> original/6(omega_mech)
  Zero-Order Hold17/1 -> original/7(theta_mech)
  Constant36/1 -> original/14(lambda_w)
  original/3(id2) -> Scope5/2
  original/5(iq2) -> Scope7/2
  Zero-Order Hold36/1 -> original2/7(theta_mech)
  Constant44/1 -> original2/12(lambda_f)
  Zero-Order Hold37/1 -> original2/3(ic)
  Constant45/1 -> original2/8(Vdc)
  Zero-Order Hold33/1 -> original2/2(ib)
  Constant42/1 -> original2/13(Tcur)
  original2/6(v_ab_out) -> Scope13/1
  Zero-Order Hold35/1 -> original2/6(omega_mech)
  original2/3(id2) -> Scope14/2
  Constant39/1 -> original2/9(Ld)
  From32/1 -> Zero-Order Hold36/1
  Gain9/1 -> Zero-Order Hold35/1
  Constant40/1 -> original2/10(Lq)
  Zero-Order Hold32/1 -> original2/1(ia)
  Constant41/1 -> original2/11(Rs)
  From29/1 -> Gain9/1
  From26/1 -> Zero-Order Hold37/1
  From27/1 -> Zero-Order Hold32/1
  original2/5(iq2) -> Scope15/2
  Constant47/1 -> Scope14/3
  Constant43/1 -> original2/14(lambda_w)
  Constant11/1 -> original2/4(id_ref)
  From28/1 -> Zero-Order Hold33/1
  Zero-Order Hold34/1 -> original2/5(iq_ref)
  From33/1 -> Zero-Order Hold34/1
  Constant2/1 -> Scope15/3
  From36/1 -> Zero-Order Hold15/1
  original2/1(gg) -> Delay One Step1/1
  original/1(gg) -> Delay One Step3/1
  f_pmsm_foc_sl/1(Out2) -> Scope8/2
  Repeating Sequence3/1 -> Manual Switch2/2
  Manual Switch2/1 -> Manual Switch6/2
  Step2/1 -> Manual Switch2/1
  Manual Switch6/1 -> Gain6/1
  [Te] -> f_pmsm_foc_sl/6(Te)
  f_pmsm_foc_sl/2(gg) -> 2levelBridge1/1
  Repeating Sequence1/1 -> Data Type Conversion8/1
  connections:
  Current Measurement1/LConn1 -- 2levelBridge1/RConn2
  Vdc/RConn1 -- 2levelBridge1/RConn1
  Current Measurement1/RConn1 -- Vdc/LConn1
  Permanent Magnet Synchronous Machine2/LConn1 -- 2levelBridge1/LConn1
  Permanent Magnet Synchronous Machine2/LConn2 -- 2levelBridge1/LConn2
  2levelBridge1/LConn3 -- Permanent Magnet Synchronous Machine2/LConn3

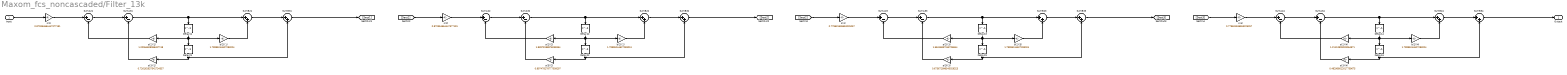
== system Maxom_fcs_noncascaded/Filter_13k ==
  Input : Inport
  Delay{11..14,21..24} (8 alike) : Delay  DelayLength=1  InitialCondition=0
  SumA{21..24,31..34} (8 alike) : Sum  Inputs=|+-  RndMeth=Nearest  SaturateOnIntegerOverflow=on  OutDataTypeStr=Inherit: Same as first input
  SumB{21..24,31..34} (8 alike) : Sum  Inputs=|++  RndMeth=Nearest  SaturateOnIntegerOverflow=on  OutDataTypeStr=Inherit: Same as first input
  a(2)(1) : Gain  Gain=1.20064608086497748  ParamDataTypeStr=double  RndMeth=Nearest  SaturateOnIntegerOverflow=on  OutDataTypeStr=Inherit: Same as input
  a(2)(2) : Gain  Gain=1.83979198876035954  ParamDataTypeStr=double  RndMeth=Nearest  SaturateOnIntegerOverflow=on  OutDataTypeStr=Inherit: Same as input
  a(2)(3) : Gain  Gain=1.58416837048726844  ParamDataTypeStr=double  RndMeth=Nearest  SaturateOnIntegerOverflow=on  OutDataTypeStr=Inherit: Same as input
  a(2)(4) : Gain  Gain=1.21113909228264971  ParamDataTypeStr=double  RndMeth=Nearest  SaturateOnIntegerOverflow=on  OutDataTypeStr=Inherit: Same as input
  a(3)(1) : Gain  Gain=0.726162637542734357  ParamDataTypeStr=double  RndMeth=Nearest  SaturateOnIntegerOverflow=on  OutDataTypeStr=Inherit: Same as input
  a(3)(2) : Gain  Gain=0.897478278777509297  ParamDataTypeStr=double  RndMeth=Nearest  SaturateOnIntegerOverflow=on  OutDataTypeStr=Inherit: Same as input
  a(3)(3) : Gain  Gain=0.673672996545029323  ParamDataTypeStr=double  RndMeth=Nearest  SaturateOnIntegerOverflow=on  OutDataTypeStr=Inherit: Same as input
  a(3)(4) : Gain  Gain=0.482908022017759675  ParamDataTypeStr=double  RndMeth=Nearest  SaturateOnIntegerOverflow=on  OutDataTypeStr=Inherit: Same as input
  b(2)(1) : Gain  Gain=1.79995244627283024  ParamDataTypeStr=double  RndMeth=Nearest  SaturateOnIntegerOverflow=on  OutDataTypeStr=Inherit: Same as input
  b(2)(2) : Gain  Gain=1.79995244627283024  ParamDataTypeStr=double  RndMeth=Nearest  SaturateOnIntegerOverflow=on  OutDataTypeStr=Inherit: Same as input
  b(2)(3) : Gain  Gain=1.79995244627283024  ParamDataTypeStr=double  RndMeth=Nearest  SaturateOnIntegerOverflow=on  OutDataTypeStr=Inherit: Same as input
  b(2)(4) : Gain  Gain=1.79995244627283024  ParamDataTypeStr=double  RndMeth=Nearest  SaturateOnIntegerOverflow=on  OutDataTypeStr=Inherit: Same as input
  s(1) : Gain  Gain=0.870354664447377191  ParamDataTypeStr=double  RndMeth=Nearest  SaturateOnIntegerOverflow=on  OutDataTypeStr=Inherit: Same as input
  s(2) : Gain  Gain=0.870354664447377191  ParamDataTypeStr=double  RndMeth=Nearest  SaturateOnIntegerOverflow=on  OutDataTypeStr=Inherit: Same as input
  s(3) : Gain  Gain=0.779631536553225257  ParamDataTypeStr=double  RndMeth=Nearest  SaturateOnIntegerOverflow=on  OutDataTypeStr=Inherit: Same as input
  s(4) : Gain  Gain=0.779631536553225257  ParamDataTypeStr=double  RndMeth=Nearest  SaturateOnIntegerOverflow=on  OutDataTypeStr=Inherit: Same as input
  Output : Outport
  wires:
  Input/1 -> s(1)/1
  s(1)/1 -> SumA21/1
  SumA21/1 -> SumA31/1
  SumA31/1 -> SumB21/1, Delay11/1
  SumB21/1 -> SumB31/1
  SumB31/1 -> [Sect1]
  a(2)(1)/1 -> SumA21/2
  Delay11/1 -> a(2)(1)/1, b(2)(1)/1, Delay21/1
  b(2)(1)/1 -> SumB21/2
  a(3)(1)/1 -> SumA31/2
  Delay21/1 -> a(3)(1)/1, SumB31/2
  [Sect1] -> s(2)/1
  s(2)/1 -> SumA22/1
  SumA22/1 -> SumA32/1
  SumA32/1 -> SumB22/1, Delay12/1
  SumB22/1 -> SumB32/1
  SumB32/1 -> [Sect2]
  a(2)(2)/1 -> SumA22/2
  Delay12/1 -> a(2)(2)/1, b(2)(2)/1, Delay22/1
  b(2)(2)/1 -> SumB22/2
  a(3)(2)/1 -> SumA32/2
  Delay22/1 -> a(3)(2)/1, SumB32/2
  [Sect2] -> s(3)/1
  s(3)/1 -> SumA23/1
  SumA23/1 -> SumA33/1
  SumA33/1 -> SumB23/1, Delay13/1
  SumB23/1 -> SumB33/1
  SumB33/1 -> [Sect3]
  a(2)(3)/1 -> SumA23/2
  Delay13/1 -> a(2)(3)/1, b(2)(3)/1, Delay23/1
  b(2)(3)/1 -> SumB23/2
  a(3)(3)/1 -> SumA33/2
  Delay23/1 -> a(3)(3)/1, SumB33/2
  [Sect3] -> s(4)/1
  s(4)/1 -> SumA24/1
  SumA24/1 -> SumA34/1
  SumA34/1 -> SumB24/1, Delay14/1
  SumB24/1 -> SumB34/1
  SumB34/1 -> Output/1
  a(2)(4)/1 -> SumA24/2
  Delay14/1 -> a(2)(4)/1, b(2)(4)/1, Delay24/1
  b(2)(4)/1 -> SumB24/2
  a(3)(4)/1 -> SumA34/2
  Delay24/1 -> a(3)(4)/1, SumB34/2

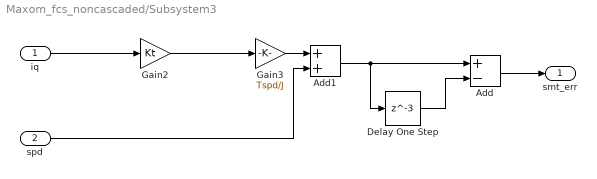
== system Maxom_fcs_noncascaded/Subsystem3 ==
  iq : Inport
  spd : Inport  Port=2
  Add : Sum  Inputs=+-
  Add1 : Sum
  Delay One Step : Delay  DelayLength=3  SampleTime=Tspd
  Gain2 : Gain  Gain=Kt
  Gain3 : Gain  Gain=Tspd/J
  smt_err : Outport
  wires:
  iq/1 -> Gain2/1
  spd/1 -> Add1/2
  Add1/1 -> Delay One Step/1, Add/1
  Delay One Step/1 -> Add/2
  Add/1 -> smt_err/1
  Gain2/1 -> Gain3/1
  Gain3/1 -> Add1/1
